simulink model "SonModel"  (R2025b)
settings: Solver=ode4  StartTime=0.0  StopTime=30  FixedStep=0.005  RelTol=1e-3
values from neighbouring files (symbols this model uses):
  CA_alpha_rad_vec = [0 2 4 5 6 7 8 9 10 11 12 13 14 15]*pi/180    [CA_RASAero_2DLUT_Gokturk_1stageVson.m]
  CA_Mach_vec = [      0.01 0.02 0.03 0.04 0.05 0.06 0.07 0.08 0.09 0.1 0.11 0.12      0.13 0.14 0.15 0.16 0.17 0.18 0.19 0.2 0.21 0.22 0.23 0.24      0.25 0.26 0.27 0.28 0.29 0.3 0.31 0.32 0.33 0.34 0.35 0.36      0.37 0.38 0.39 0.4 0.41 0.42 0.43 0.44 0.45 0.46 0.47 0.48      0.49 0.5 0.51 0.52 0.53 0.54 0.55 0.56 0.57 0.58 0.59 0.6      0.61 0.62 0.63 0.64 0.65 0.66 0.67 0.68 0.69 0.7 0.71 0.72      0.73 0.74  ...(+14344 chars)    [CA_RASAero_2DLUT_Gokturk_1stageVson.m]
  CA_table = [ ... (first row only)    [CA_RASAero_2DLUT_Gokturk_1stageVson.m]
  CN_alpha_rad_vec = [0 2 4 5 6 7 8 9 10 11 12 13 14 15]*pi/180    [CN_RASAero_2DLUT_Gokturk_1stageVson.m]
  CN_Mach_vec = [      0.01 0.02 0.03 0.04 0.05 0.06 0.07 0.08 0.09 0.1 0.11 0.12      0.13 0.14 0.15 0.16 0.17 0.18 0.19 0.2 0.21 0.22 0.23 0.24      0.25 0.26 0.27 0.28 0.29 0.3 0.31 0.32 0.33 0.34 0.35 0.36      0.37 0.38 0.39 0.4 0.41 0.42 0.43 0.44 0.45 0.46 0.47 0.48      0.49 0.5 0.51 0.52 0.53 0.54 0.55 0.56 0.57 0.58 0.59 0.6      0.61 0.62 0.63 0.64 0.65 0.66 0.67 0.68 0.69 0.7 0.71 0.72      0.73 0.74  ...(+14344 chars)    [CN_RASAero_2DLUT_Gokturk_1stageVson.m]
  CN_table = [ ... (first row only)    [CN_RASAero_2DLUT_Gokturk_1stageVson.m]
  CP_alpha_rad_vec = [0 2 4 5 6 7 8 9 10 11 12 13 14 15]*pi/180    [CP_RASAero_2DLUT_Gokturk_1stageVson.m]
  CP_Mach_vec = [      0.01 0.02 0.03 0.04 0.05 0.06 0.07 0.08 0.09 0.1 0.11 0.12      0.13 0.14 0.15 0.16 0.17 0.18 0.19 0.2 0.21 0.22 0.23 0.24      0.25 0.26 0.27 0.28 0.29 0.3 0.31 0.32 0.33 0.34 0.35 0.36      0.37 0.38 0.39 0.4 0.41 0.42 0.43 0.44 0.45 0.46 0.47 0.48      0.49 0.5 0.51 0.52 0.53 0.54 0.55 0.56 0.57 0.58 0.59 0.6      0.61 0.62 0.63 0.64 0.65 0.66 0.67 0.68 0.69 0.7 0.71 0.72      0.73 0.74  ...(+14344 chars)    [CP_RASAero_2DLUT_Gokturk_1stageVson.m]
  CP_table = [ ... (first row only)    [CP_RASAero_2DLUT_Gokturk_1stageVson.m]
undefined symbols (not defined in the file or in its folder): Cg, dCA_table, dCm_table, dCN_table, delta_max, g, I_total, KTS_alpha_rad_vec, KTS_delta_rad_vec, KTS_Mach_vec, m_propellant, m_rocket, servo_rate, servo_tau, Sref, thrust, time, time2
libraries: simulink_extras x7, simulink x3, aerolibobsolete x1, slpidlib x1, aerolibatmos2 x1
(part 2 of 2)

== matlab function SonModel/MATLAB Function11 ==
  data: V_ground_b input; V_air_b output; DCM_be input; V_wind_b output; V_air_mag output
function [V_air_b, V_wind_b, V_air_mag] = WindRelativeVelocity_OpenRocket(V_ground_b, DCM_be)
%#codegen
% GOKTURK 1stageVson: CONSTANT WIND matching OpenRocket test
%
% OpenRocket launch settings:
%   Average wind speed: 6 m/s
%   Wind direction: 90 deg (FROM EAST)
%   Std. deviation: 0 m/s (steady wind test)
%   Turbulence: 0 %
%
% Frame: Earth NED: +X North, +Y East, +Z Down.
%        Body: +X Forward, +Y Right, +Z Down.
%
% IMPORTANT: To make the rocket's longitudinal/pitch plane align
% with the OpenRocket rail pointing INTO this east wind, set the
% initial yaw (psi) in the 6DOF block to +90 deg.
% Keep the rail's velocity/position signals as GROUND velocities.
% Only aerodynamic calculations should use V_air_b.
%
% Input V_ground_b: 6DOF 'Vb' output (3x1), rocket/ground velocity in body axes.
% Input DCM_be: 6DOF 'DCMbe' output (3x3), Earth NED -> body axes.
%
% Output V_air_b: true velocity of rocket relative to the air in body axes.
% Output V_wind_b: wind velocity in body axes.
% Output V_air_mag: airspeed magnitude in m/s for Mach = V_air_mag/a.

wind_speed_mps = 6.0;
wind_from_deg = 0.0;

% Wind direction is where the wind COMES FROM.
% In NED, wind blowing FROM the East points toward the West:
wind_from_rad = wind_from_deg * pi / 180.0;
V_wind_e = [-wind_speed_mps*cos(wind_from_rad);
            -wind_speed_mps*sin(wind_from_rad);
             0.0];

% Earth -> body rotation, from 6DOF output.
V_wind_b = DCM_be * V_wind_e;

% Relative velocity for aerodynamic coefficients and qbar.
V_air_b = V_ground_b - V_wind_b;

V_air_mag = sqrt(V_air_b(1)^2 + V_air_b(2)^2 + V_air_b(3)^2);
end

== matlab function SonModel/MATLAB Function12 ==
  settings: updateMethod=DISCRETE  sampleTime=0.01
  data: delta_des_deg input; delta_servo_deg output; active input; delta_ff_deg output; comp_limited output

function [delta_servo_deg, delta_ff_deg, comp_limited] = ...
    Servo_Comp_DI(delta_des_deg, active)
%#codegen

% INPUTS
% delta_des_deg : Desired elevator angle [deg]
% active        : Allocation enabled (0/1)

% OUTPUTS
% delta_servo_deg : Servo input command [deg]
% delta_ff_deg    : Added feedforward [deg]
% comp_limited    : Compensation saturation flag

persistent delta_prev rate_filtered was_active

if isempty(was_active)
    delta_prev = 0.0;
    rate_filtered = 0.0;
    was_active = false;
end

%% PARAMETERS

Ts = 0.01;

servo_tau = 0.05;

% Derivative low-pass filter time constant
tau_filter = 0.04;

% Maximum actuator angle [deg]
delta_max = 15.0;

% Allocation internal rate limit [deg/s]
rate_max = 30.0;

%% OUTPUT INITIALIZATION

delta_servo_deg = 0.0;
delta_ff_deg = 0.0;
comp_limited = false;

%% VALIDITY AND RESET

valid = (active ~= 0) && isfinite(delta_des_deg);

if ~valid
    delta_prev = 0.0;
    rate_filtered = 0.0;
    was_active = false;
    return;
end

%% DESIRED DEFLECTION

delta_des = min(max( ...
    delta_des_deg,-delta_max),delta_max);

% Prevent derivative kick at activation
if ~was_active
    delta_prev = delta_des;
    rate_filtered = 0.0;
    was_active = true;
end

%% DESIRED DEFLECTION RATE

delta_rate = (delta_des-delta_prev)/Ts;

% Numerical robustness
delta_rate = min(max( ...
    delta_rate,-rate_max),rate_max);

%% FILTER THE DERIVATIVE

a = Ts/(tau_filter+Ts);

rate_filtered = rate_filtered + ...
    a*(delta_rate-rate_filtered);

%% SERVO DYNAMIC COMPENSATION

delta_ff_deg = servo_tau*rate_filtered;

delta_unlimited = delta_des + delta_ff_deg;

%% FINAL ANGLE SATURATION

delta_servo_deg = min(max( ...
    delta_unlimited,-delta_max),delta_max);

comp_limited = ...
    abs(delta_servo_deg-delta_unlimited) > 1e-9;

%% UPDATE STATE

delta_prev = delta_des;

end

== matlab function SonModel/MATLAB Function19 ==
  settings: updateMethod=DISCRETE  sampleTime=0.01
  data: t input; h_ref output; thrust input; x input; h input; gamma input; gamma_ref output; active output; blend output; cutoff_state output; path_valid output
function [h_ref, gamma_ref, active, blend, cutoff_state, path_valid] = ...
    Reference_Trajectory(t, thrust, x, h, gamma)
%#codegen
% Reference generator for a single-burn, forward-moving X-h simulation.
% Paste the entire file into a Simulink MATLAB Function block.
% Update method: Discrete; initial sample time: 0.01 s.
%
% INPUTS (scalar doubles)
% t       : time [s]
% thrust  : nonnegative engine thrust magnitude [N], NOT net body force
% x       : signed horizontal displacement from launch [m]
% h       : height above target ground plane [m], positive upward
% gamma   : atan2(-Vz_earth, Vx_earth) [rad], X-h projected path angle
%
% OUTPUTS
% h_ref, gamma_ref : geometric path references [m, rad]
% active          : controller enable (boolean)
% blend           : enable weight, smooth 0-to-1 transition
% cutoff_state    : [detected time (s), x (m), h (m), gamma (rad)]
%                   time = -1 means cutoff has not been detected
% path_valid      : captured endpoint geometry passes basic checks
%
% This is NOT an elevator controller or a feasibility/landing guarantee.
% Assumes one burn, negligible lateral motion, and increasing x.
% gamma_f and blend_time are initial experiment settings, not tuned values.
% For separate MATLAB runs, use: clear Reference_Trajectory

persistent motor_seen captured finished tb xb hb gb

if isempty(captured)
    motor_seen = false;
    captured = false;
    finished = false;
    tb = -1.0;
    xb = 0.0;
    hb = 0.0;
    gb = 0.0;
end

xf = 3000.0;
hf = 0.0;
gamma_f = -45.0*pi/180.0;
thrust_eps = 1.0e-6; % ideal simulation signal; not a noise filter
blend_time = 0.30;   % s; tune with the subsequent controller

h_ref = h;
gamma_ref = gamma;
active = false;
blend = 0.0;
path_valid = false;

% Arm only after observing nonzero thrust. Latch the first cutoff once.
if ~captured
    if thrust > thrust_eps
        motor_seen = true;
    elseif motor_seen && abs(thrust) <= thrust_eps
        tb = t;
        xb = x;
        hb = h;
        gb = gamma;
        captured = true;
    end
end

cutoff_state = [tb, xb, hb, gb];
if ~captured
    return;
end

L = xf - xb;
if L <= 1.0 || hb <= hf || abs(gb) >= 85.0*pi/180.0
    return;
end

% Cubic Hermite polynomial with terminal height = 0.
m0 = tan(gb);
mf = tan(gamma_f);
a0 = hb;
a1 = L*m0;
a2 = 3.0*(hf-hb) - L*(2.0*m0+mf);
a3 = 2.0*(hb-hf) + L*(m0+mf);

% Check that the cubic stays above ground before the target.
% For hf=0, h(s)=(1-s)*Q(s); check the minimum of quadratic Q.
q0 = hb;
q1 = hb + L*m0;
q2 = -a3;
qmin = min(q0, -L*mf);
if q2 > 0.0
    sv = -q1/(2.0*q2);
    if sv > 0.0 && sv < 1.0
        qmin = min(qmin, q0 + q1*sv + q2*sv*sv);
    end
end
if qmin <= 0.0
    return;
end
path_valid = true;

% Stop enabling after ground contact; reaching x=xf alone does not disable.
if h <= hf
    finished = true;
end
if finished
    h_ref = hf;
    gamma_ref = gamma_f;
    return;
end

s = (x-xb)/L;
if s < 0.0
    h_ref = hb + m0*(x-xb);
    gamma_ref = gb;
elseif s <= 1.0
    h_ref = a0 + a1*s + a2*s*s + a3*s*s*s;
    dhdx = (a1 + 2.0*a2*s + 3.0*a3*s*s)/L;
    gamma_ref = atan(dhdx);
else
    % Mathematical continuation only: avoid a sudden disable at x=3000.
    % Being airborne here means the terminal target has been missed.
    h_ref = hf + mf*(x-xf);
    gamma_ref = gamma_f;
end

r = min(max((t-tb)/blend_time, 0.0), 1.0);
blend = r*r*(3.0-2.0*r);
active = true;
end

== matlab function SonModel/Inertia of Moment Bloğu/MATLAB Function1 ==
  data: Ixxx input; I_matrix output; Iyyy input; Izzz input
function I_matrix = inertia_matrix(Ixxx, Iyyy, Izzz)

% Ixxx, Iyyy, Izzz: anlık atalet momentleri [kg*m^2]
% Çıkış: 6DOF bloğuna verilecek 3x3 inertia tensor matrisi

I_matrix = zeros(3,3);

I_matrix(1,1) = Ixxx;
I_matrix(2,2) = Iyyy;
I_matrix(3,3) = Izzz;

end

== matlab function SonModel/MATLAB Function20 ==
  data: h_ref input; gamma_cmd output; gamma_ref input; h input; gamma input; active input; e_h output
function [gamma_cmd, e_h] = Path_Guidance(h_ref, gamma_ref, h, gamma, active)
%#codegen
% Inputs/outputs: heights [m], angles [rad]. No persistent state.
% Initial geometric guidance settings; NOT tuned for the user's aircraft.
lookahead = 500.0;          % m; larger = weaker height-error correction
correction_max = 10*pi/180;
gamma_min = -80*pi/180;
gamma_max = 80*pi/180;
e_h = h_ref - h;
gamma_cmd = gamma;
if active
    correction = atan2(e_h, lookahead);
    correction = min(max(correction, -correction_max), correction_max);
    gamma_cmd = min(max(gamma_ref + correction, gamma_min), gamma_max);
end
end

== matlab function SonModel/MATLAB Function21 ==
  settings: updateMethod=DISCRETE  sampleTime=0.01
  data: qdot_cmd input; delta_e_deg output; Iyy input; Cm0 input; uair input; wair input; rho input; Sref input; cbar input; My_damping input; dCm_curve input; active input; blend input; My_cmd output; dCm_req output; dCm_applied output; limited output; enabled output
function [delta_e_deg, My_cmd, dCm_req, dCm_applied, limited, enabled] = ...
    Moment_Allocation_DI(qdot_cmd, Iyy, Cm0, uair, wair, rho, ...
                         Sref, cbar, My_damping, dCm_curve, active, blend)
%#codegen
% 2D X-Z-pitch simulation: two elevators share ONE deflection command.
%
% Inputs:
% qdot_cmd     [rad/s^2] commanded pitch angular acceleration
% Iyy          [kg*m^2] pitch moment of inertia
% Cm0          [-] base pitch-moment coefficient (delta_e = 0)
% uair, wair   [m/s] AIR-RELATIVE body X and Z velocity components
% rho          [kg/m^3] atmospheric density
% Sref         [m^2] reference area
% cbar         [m] pitch moment reference chord
% My_damping   [N*m] baseline pitch damping and any other base moment;
%                    connect Constant(0) if no such contribution exists
% dCm_curve    [7x1] Delta Cm at delta_e = -15,-10,-5,0,5,10,15 deg
% active       logical: guidance / model / LUT validity allow control
% blend        [0,1] ramp after engine cutoff
%
% NOTE: body X/Z air-relative, not NED ground speed. For strict 2D v_air=0.
% NOTE: do not double-count the two elevators if the DeltaCm data already
%       represent the combined surfaces.
% NOTE: positive pitch moment sign must match the actual 6DoF axes.

persistent delta_prev
if isempty(delta_prev)
    delta_prev = 0.0;
end

Ts = 0.01;        % Must match block's DISCRETE execution period [s]
deg_grid = [-15.0, -10.0, -5.0, 0.0, 5.0, 10.0, 15.0];
delta_max = 15.0; % deg
rate_max  = 30.0; % deg/s; demonstration value, replace if measured
small = 1e-12;

% Internally calculate dynamic pressure and base pitching moment.
Va = hypot(uair, wair);
qbar = 0.5 * rho * Va * Va;
moment_scale = qbar * Sref * cbar;   % [N*m] per Cm
My_base = moment_scale * Cm0 + My_damping;
My_cmd = Iyy * qdot_cmd;

dCm_req = 0.0;
dCm_applied = 0.0;
delta_e_deg = 0.0;
enabled = (active ~= 0) && Iyy > 0.0 && ...
    moment_scale > 1e-6 && Va > 1.0 && ...
    isfinite(My_cmd) && isfinite(My_base) && ...
    all(isfinite(dCm_curve));

if ~enabled
    delta_prev = 0.0;
    limited = (active ~= 0);
    return;
end

dCm_req = (My_cmd - My_base) / moment_scale;

% Piecewise inverse of the original DeltaCm-vs-deflection curve.
% If several deflections produce the requested DeltaCm, select the
% solution nearest the previously commanded deflection.
found = false;
best_delta = 0.0;
best_move = Inf;

for i = 1:6
    c1 = dCm_curve(i);
    c2 = dCm_curve(i+1);
    if dCm_req >= min(c1,c2)-small && dCm_req <= max(c1,c2)+small
        if abs(c2-c1) < small
            candidate = min(max(delta_prev,deg_grid(i)),deg_grid(i+1));
        else
            lambda = (dCm_req - c1)/(c2 - c1);
            lambda = min(max(lambda,0.0),1.0);
            candidate = deg_grid(i) + ...
                lambda*(deg_grid(i+1)-deg_grid(i));
        end
        move = abs(candidate-delta_prev);
        if ~found || move < best_move
            found = true;
            best_move = move;
            best_delta = candidate;
        end
    end
end

% Requested moment is outside the achievable curve: choose the best
% available tabulated deflection, and flag saturation.
if ~found
    best_error = Inf;
    best_move = Inf;
    for i = 1:7
        err = abs(dCm_req - dCm_curve(i));
        move = abs(deg_grid(i)-delta_prev);
        if err < best_error-small || ...
           (abs(err-best_error) <= small && move < best_move)
            best_error = err;
            best_move = move;
            best_delta = deg_grid(i);
        end
    end
end

% Smooth engagement + rate/angle limits.
weight = min(max(blend,0.0),1.0);
delta_target = min(max(weight*best_delta,-delta_max),delta_max);
max_step = rate_max*Ts;
step = min(max(delta_target-delta_prev,-max_step),max_step);
delta_e_deg = min(max(delta_prev+step,-delta_max),delta_max);
delta_prev = delta_e_deg;

% Estimate the DeltaCm actually requested after limits.
dCm_applied = dCm_curve(7);
for i = 1:6
    if delta_e_deg <= deg_grid(i+1)
        lambda = (delta_e_deg-deg_grid(i)) / ...
                 (deg_grid(i+1)-deg_grid(i));
        dCm_applied = dCm_curve(i) + ...
            lambda*(dCm_curve(i+1)-dCm_curve(i));
        break;
    end
end
limited = ~found || abs(dCm_applied-dCm_req) > 1e-5;
end

== matlab function SonModel/Inertia of Moment Bloğu/MATLAB Function ==
  data: Ixx_dry input; Ixx output; Iyy_dry input; Izz_dry input; dIxx input; dIyy input; dIzz input; m_burned input; m_propellant input; Iyy output; Izz output
function [Ixx, Iyy, Izz] = inertia_update( ...
    Ixx_dry, Iyy_dry, Izz_dry, ...
    dIxx, dIyy, dIzz, ...
    m_burned, m_propellant)

% m_burned      : o ana kadar yanan yakıt kütlesi [kg]
% m_propellant  : toplam propellant kütlesi [kg]
%
% Denklem:
% oran = 1 - m_burned / m_propellant
% I(t) = I_dry + oran * dI

if m_propellant > 0
    oran = 1 - m_burned / m_propellant;
else
    oran = 0;
end

% oranı 0-1 arasında sınırla
if oran < 0
    oran = 0;
elseif oran > 1
    oran = 1;
end

Ixx = Ixx_dry + oran * dIxx;
Iyy = Iyy_dry + oran * dIyy;
Izz = Izz_dry + oran * dIzz;

end

== matlab function SonModel/Inertia of Moment Bloğu/MATLAB Function2 ==
  data: dIxx input; dI_dt_matrix output; dIyy input; dIzz input; m_dot input; m_propellant input
function dI_dt_matrix = inertia_dot_matrix(dIxx, dIyy, dIzz, m_dot, m_propellant)

% dIxx, dIyy, dIzz : wet - dry inertia farkları [kg*m^2]
% m_dot            : pozitif yakıt tüketim hızı [kg/s]
% m_propellant     : toplam propellant kütlesi [kg]
%
% Çıkış:
% dI_dt_matrix     : 6DOF dI/dt girişine verilecek 3x3 matris

if m_propellant > 0
    oran_dot = -m_dot / m_propellant;
else
    oran_dot = 0;
end

Ixx_dot = oran_dot * dIxx;
Iyy_dot = oran_dot * dIyy;
Izz_dot = oran_dot * dIzz;

dI_dt_matrix = [Ixx_dot  0        0;
                0        Iyy_dot  0;
                0        0        Izz_dot];

end

== matlab function SonModel/MATLAB Function ==
  data: u_rel input; alpha_signed_rad output; w_rel input; alpha_RASAero_rad output
function [alpha_signed_rad, alpha_RASAero_rad] = calc_alpha_3DOF(u_rel, w_rel)

V = sqrt(u_rel^2 + w_rel^2);

% Cok dusuk hizlarda AoA anlamli degil
if V < 1.0
    alpha_signed_rad  = 0;
    alpha_RASAero_rad = 0;
    return;
end

%% Gercek signed AoA
alpha_signed_rad = atan2(w_rel, u_rel);

%% RASAero LUT icin |AoA|
alpha_RASAero_rad = abs(alpha_signed_rad);

%% RASAero veri siniri = 15 derece
alpha_max = 15*pi/180;

if alpha_RASAero_rad > alpha_max
    alpha_RASAero_rad = alpha_max;
end

end

== matlab function SonModel/MATLAB Function1 ==
  data: CA input; rho input; u input; v input; F_aero_b output; w input; Sref input

function F_aero_b = CA_to_Fdrag_body_3DOF(CA, rho, u, v, w, Sref)

%#codegen

% GOKTURK - Axial Aerodynamic Force
%
% CA   : Total axial force coefficient
%        CA = CA_RASAero + DeltaCA_canard
%
% rho  : Air density [kg/m^3]
% u,v,w: Air-relative body velocities [m/s]
% Sref : Reference area [m^2]
%
% Body axes:
% +X : Forward
% +Y : Right
% +Z : Down

%% 1) Total air-relative speed
V_air = sqrt(u^2 + v^2 + w^2);

if V_air < 1e-6
    F_aero_b = [0; 0; 0];
    return;
end

%% 2) Dynamic pressure
qbar = 0.5 * rho * V_air^2;

%% 3) Axial aerodynamic force
Fx = -qbar * Sref * CA;

%% 4) Body-frame force vector
F_aero_b = [Fx;
            0;
            0];

end

== matlab function SonModel/MATLAB Function2 ==
  data: CN input; rho input; Sref input; u input; v input; F_normal_b output; w input; CG_m input; CP_m input; M_aero_b output

function [F_normal_b, M_aero_b] = aero_CN_CP_moment_3DOF( ...
    CN, rho, Sref, u, v, w, CG_m, CP_m)

%#codegen

% Body axes:
% +X : Forward
% +Y : Right
% +Z : Down
%
% u, v, w : Air-relative body velocities [m/s]
%
% CN : Signed pitch-plane normal force coefficient
%
% Calculates:
% Fz : Pitch-plane normal force
% My : Pitching moment about CG

%% 1) Total air-relative speed

V = sqrt(u^2 + v^2 + w^2);

if V < 1e-6
    F_normal_b = [0; 0; 0];
    M_aero_b   = [0; 0; 0];
    return;
end

%% 2) Dynamic pressure

qbar = 0.5 * rho * V^2;

%% 3) Pitch-plane normal force

Fz = -qbar * Sref * CN;

F_normal_b = [0;
              0;
              Fz];

%% 4) Pitching moment about CG

% CG and CP measured from rocket nose [m]

x_arm = CG_m - CP_m;

My = -x_arm * Fz;

M_aero_b = [0;
            My;
            0];

end

== matlab function SonModel/MATLAB Function3 ==
  settings: updateMethod=DISCRETE  sampleTime=0.01
  data: gamma_cmd input; qdot_cmd output; gamma_gnd input; theta_hat input; alpha_hat input; q_hat input; uair input; wair input; active input; q_ref output; theta_ref output; alpha_cmd output; e_gamma output; enabled output

function [qdot_cmd, q_ref, theta_ref, alpha_cmd, e_gamma, enabled] = ...
    Attitude_Rate_DI(gamma_cmd, gamma_gnd, theta_hat, ...
                     alpha_hat, q_hat, uair, wair, active)
%#codegen

% INPUTS:
% gamma_cmd : Target ground flight path angle [rad]
% gamma_gnd : Actual ground flight path angle [rad]
% theta_hat : Pitch angle [rad]
% alpha_hat : Angle of attack [rad]
% q_hat     : Pitch angular velocity [rad/s]
% uair      : Air-relative body X velocity [m/s]
% wair      : Air-relative body Z velocity [m/s]
% active    : Controller enable (0/1)

% OUTPUTS:
% qdot_cmd  : Desired pitch acceleration [rad/s^2]
% q_ref     : Desired pitch rate [rad/s]
% theta_ref : Desired pitch angle [rad]
% alpha_cmd : Desired AoA [rad]
% e_gamma   : Flight path tracking error [rad]
% enabled   : Controller status

persistent alpha_base rate_integral was_active

if isempty(was_active)
    alpha_base = 0.0;
    rate_integral = 0.0;
    was_active = false;
end

%% 1. SAMPLE TIME

Ts = 0.01;

%% 2. CONTROLLER GAINS

Kgamma = 0.45;

% UPDATED: Stronger AoA tracking response
Ktheta = 1.5;      % Previous value: 1.0

Kp_rate = 1.8;
Ki_rate = 0.0;

%% 3. LIMITS

alpha_min = -5*pi/180;
alpha_max =  7*pi/180;

q_ref_max = 20*pi/180;
qdot_max = 25*pi/180;

integral_max = 5*pi/180;

%% 4. AIR-RELATIVE VARIABLES

Va = hypot(uair, wair);

gamma_air = theta_hat - alpha_hat;

%% 5. INITIALIZE OUTPUTS

qdot_cmd = 0.0;
q_ref = 0.0;

theta_ref = theta_hat;
alpha_cmd = alpha_hat;

e_gamma = atan2( ...
    sin(gamma_cmd-gamma_gnd), ...
    cos(gamma_cmd-gamma_gnd));

enabled = (active ~= 0) && ...
          isfinite(Va) && ...
          isfinite(gamma_cmd) && ...
          isfinite(gamma_gnd) && ...
          isfinite(theta_hat) && ...
          isfinite(alpha_hat) && ...
          isfinite(q_hat) && ...
          Va > 5.0;

if ~enabled
    rate_integral = 0.0;
    was_active = false;
    return;
end

%% 6. INITIALIZE AT ACTIVATION

if ~was_active

    alpha_base = min(max( ...
        alpha_hat,alpha_min),alpha_max);

    rate_integral = 0.0;

    was_active = true;
end

%% 7. FLIGHT PATH CONTROLLER

alpha_cmd = alpha_base + Kgamma*e_gamma;

alpha_cmd = min(max( ...
    alpha_cmd,alpha_min),alpha_max);

%% 8. PITCH / AOA CONTROLLER

theta_ref = gamma_air + alpha_cmd;

e_theta = atan2( ...
    sin(theta_ref-theta_hat), ...
    cos(theta_ref-theta_hat));

% UPDATED: Ktheta = 1.5
q_ref = Ktheta*e_theta;

q_ref = min(max( ...
    q_ref,-q_ref_max),q_ref_max);

%% 9. PITCH RATE CONTROLLER

e_rate = q_ref-q_hat;

raw_qdot = Kp_rate*e_rate + ...
           Ki_rate*rate_integral;

qdot_cmd = min(max( ...
    raw_qdot,-qdot_max),qdot_max);

%% 10. INTEGRAL ANTI-WINDUP

if abs(raw_qdot) < qdot_max || ...
   raw_qdot*e_rate < 0

    rate_integral = min(max( ...
        rate_integral + Ts*e_rate, ...
        -integral_max),integral_max);

end

end
